simulink model "DAB_Controller_PIL"  (R2025b)
settings: Solver=FixedStepDiscrete  StartTime=0.0  StopTime=inf  FixedStep=1e-7  RelTol=1e-3
settings Model: Creator=vivid  LastModifiedBy=vivid
settings DataIOCC: SaveOutput=off  SignalLogging=off  DSMLogging=off  StreamToWks=off  SaveTime=off  ReturnWorkspaceOutputs=off
settings OptimizationCC: DefaultParameterBehavior=Inlined  EnhancedBackFolding=on  PassReuseOutputArgsAs=Individual arguments  ZeroExternalMemoryAtStartup=off  ZeroInternalMemoryAtStartup=off  MaxStackSize=512  OptimizeBlockOrder=speed  DifferentSizesBufferReuse=on  OptimizationCustomize=off  EfficientTunableParamExpr=on
settings DebuggingCC: ParameterTunabilityLossMsg=error
settings HardwareCC: ProdBitPerPointer=32.0  ProdBitPerSizeT=32.0  ProdBitPerPtrDiffT=32.0  ProdLargestAtomicInteger=Long  ProdLargestAtomicFloat=Double  ProdWordSize=32.0  ProdLongLongMode=on  ProdHWDeviceType=ARM Compatible->ARM Cortex-M
settings SFSimCC: MATLABDynamicMemAlloc=off
settings RTWCC: SystemTargetFile=ert.tlc  HardwareBoard=STM32G4xx Based  TemplateMakefile=ert_default_tmf  Toolchain=GNU Tools for ARM Embedded Processors  Description=Embedded Coder
settings CodeAppCC: ForceParamTrailComments=on  IgnoreCustomStorageClasses=off  MaxIdLength=63.0  OperatorAnnotations=on  SimulinkDataObjDesc=on  SFDataObjDesc=on  InsertBlockDesc=on
settings ERTTargetCC: ExtModeTransport=3.0  ExtModeStaticAlloc=on  ExtModeStaticAllocSize=2048.0  ExtModeMexFile=ext_xcp  ExtModeIntrfLevel=Level2 - Open  RootIOFormat=Structure reference  TargetLangStandard=C99 (ISO)  CodeReplacementLibrary=ARM Cortex-M  SupportAbsoluteTime=off  SupportNonFinite=off

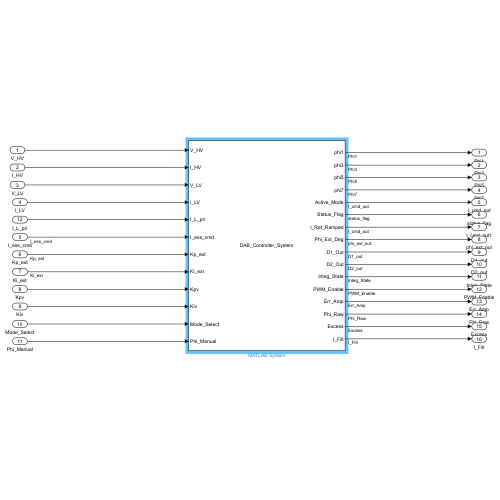
[thumbnail: Simulink's stored preview of the top-level diagram]
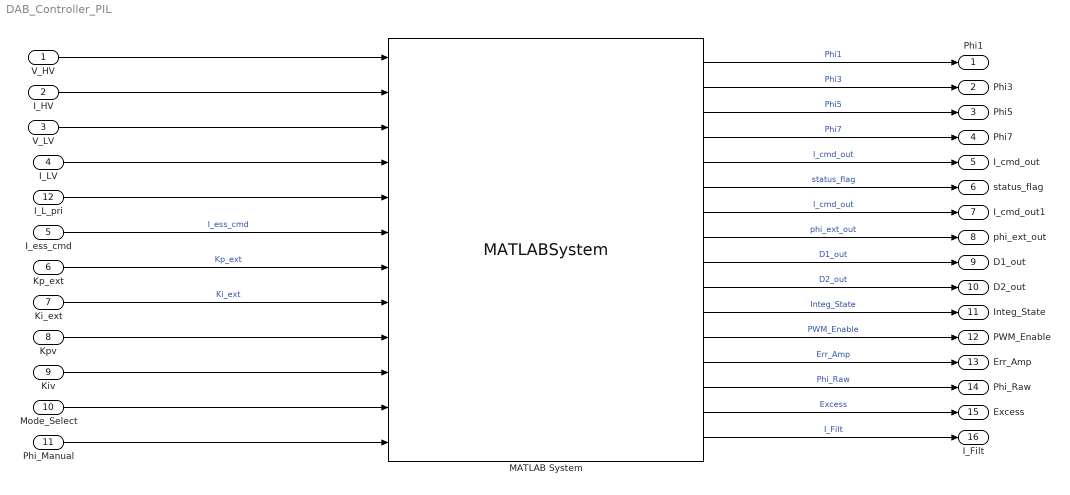
== system DAB_Controller_PIL ==
  V_HV : Inport  OutDataTypeStr=double  PortDimensions=1  SampleTime=1e-7
  I_HV : Inport  Port=2  OutDataTypeStr=double  PortDimensions=1  SampleTime=1e-7
  V_LV : Inport  Port=3  OutDataTypeStr=double  PortDimensions=1  SampleTime=1e-7
  I_LV : Inport  Port=4  OutDataTypeStr=double  PortDimensions=1  SampleTime=1e-7
  I_ess_cmd : Inport  Port=5  OutDataTypeStr=double  PortDimensions=[1 1]  SampleTime=1e-7
  Kp_ext : Inport  Port=6  OutDataTypeStr=double  PortDimensions=[1 1]  SampleTime=1e-7
  Ki_ext : Inport  Port=7  OutDataTypeStr=double  PortDimensions=[1 1]  SampleTime=1e-7
  Kpv : Inport  Port=8  OutDataTypeStr=double  PortDimensions=1  SampleTime=1e-7
  Kiv : Inport  Port=9  OutDataTypeStr=double  PortDimensions=1  SampleTime=1e-7
  Mode_Select : Inport  Port=10  OutDataTypeStr=double  PortDimensions=1  SampleTime=1e-7
  Phi_Manual : Inport  Port=11  OutDataTypeStr=double  PortDimensions=1  SampleTime=1e-7
  I_L_pri : Inport  Port=12  OutDataTypeStr=double  PortDimensions=1  SampleTime=1e-7
  MATLAB System : MATLABSystem  System=DAB_Controller_System  Fs=80e3  Ts_ctrl=1e-7  L_leakage=90e-6  SPS_Inner_Phase=180  InitDelay=0.0001  V_HV_Ref=380  V_HV_Band=30  I_ESS_Max=10  I_UPS_Max=30  V_Pack_Max=109.2  V_CV_Start=108.0  K_CV=5.0  V_ESS_Limit=93.0  V_UPS_Limit=87.0  V_Min_Limit=84.0  EnableFF=true  SoftStartTime=0.0002  MaxSlewRate=1e5  MaxPhaseRate=1e5  DeadZone=0  GainSched_Threshold=2.0  GainSched_Factor=1.0  EnableFluxBalancing=true  Flux_Kp=0.005  Flux_Ki=0.05  Flux_Limit=0.02  SimulateUsing=Code generation
      mask Type: DAB_Controller_System
  Phi1 : Outport  OutDataTypeStr=double  PortDimensions=[1 1]  SampleTime=1e-7
  Phi3 : Outport  Port=2  OutDataTypeStr=double  PortDimensions=[1 1]  SampleTime=1e-7
  Phi5 : Outport  Port=3  OutDataTypeStr=double  PortDimensions=[1 1]  SampleTime=1e-7
  Phi7 : Outport  Port=4  OutDataTypeStr=double  PortDimensions=[1 1]  SampleTime=1e-7
  I_cmd_out : Outport  Port=5  OutDataTypeStr=double  PortDimensions=[1 1]  SampleTime=1e-7
  status_flag : Outport  Port=6  OutDataTypeStr=double  PortDimensions=[1 1]  SampleTime=1e-7
  I_cmd_out1 : Outport  Port=7  OutDataTypeStr=double  PortDimensions=[1 1]  SampleTime=1e-7
  phi_ext_out : Outport  Port=8  OutDataTypeStr=double  PortDimensions=[1 1]  SampleTime=1e-7
  D1_out : Outport  Port=9  OutDataTypeStr=double  PortDimensions=[1 1]  SampleTime=1e-7
  D2_out : Outport  Port=10  OutDataTypeStr=double  PortDimensions=[1 1]  SampleTime=1e-7
  Integ_State : Outport  Port=11  OutDataTypeStr=double  PortDimensions=[1 1]  SampleTime=1e-7
  PWM_Enable : Outport  Port=12  OutDataTypeStr=double  PortDimensions=[1 1]  SampleTime=1e-7
  Err_Amp : Outport  Port=13  OutDataTypeStr=double  PortDimensions=[1 1]  SampleTime=1e-7
  Phi_Raw : Outport  Port=14  OutDataTypeStr=double  PortDimensions=[1 1]  SampleTime=1e-7
  Excess : Outport  Port=15  OutDataTypeStr=double  PortDimensions=[1 1]  SampleTime=1e-7
  I_Filt : Outport  Port=16  OutDataTypeStr=double  PortDimensions=[1 1]  SampleTime=1e-7
  wires:
  V_HV/1 -> MATLAB System/1
  MATLAB System/1 -> Phi1/1  "Phi1"
  MATLAB System/8 -> phi_ext_out/1  "phi_ext_out"
  MATLAB System/9 -> D1_out/1  "D1_out"
  MATLAB System/5 -> I_cmd_out/1  "I_cmd_out"
  MATLAB System/7 -> I_cmd_out1/1  "I_cmd_out"
  Ki_ext/1 -> MATLAB System/8  "Ki_ext"
  I_HV/1 -> MATLAB System/2
  Kpv/1 -> MATLAB System/9
  MATLAB System/4 -> Phi7/1  "Phi7"
  Kiv/1 -> MATLAB System/10
  MATLAB System/3 -> Phi5/1  "Phi5"
  MATLAB System/10 -> D2_out/1  "D2_out"
  V_LV/1 -> MATLAB System/3
  I_LV/1 -> MATLAB System/4
  Kp_ext/1 -> MATLAB System/7  "Kp_ext"
  MATLAB System/11 -> Integ_State/1  "Integ_State"
  MATLAB System/6 -> status_flag/1  "status_flag"
  MATLAB System/2 -> Phi3/1  "Phi3"
  I_ess_cmd/1 -> MATLAB System/6  "I_ess_cmd"
  MATLAB System/16 -> I_Filt/1  "I_Filt"
  MATLAB System/15 -> Excess/1  "Excess"
  MATLAB System/14 -> Phi_Raw/1  "Phi_Raw"
  MATLAB System/12 -> PWM_Enable/1  "PWM_Enable"
  MATLAB System/13 -> Err_Amp/1  "Err_Amp"
  Phi_Manual/1 -> MATLAB System/12
  Mode_Select/1 -> MATLAB System/11
  I_L_pri/1 -> MATLAB System/5
